simulink model "AlKaseeh_PhysicalTwin_PM_FinalScientific_v4_6_2"  (R2025b)
settings: Solver=ode15s  StartTime=0.0  StopTime=9000  MaxStep=0.1  RelTol=1e-4
libraries: fl_lib x34, nesl_utility x24, ee_lib x1, slpidlib x1, SimscapeFluids_lib x1
(part 1 of 2)
settings Model: Creator=Iman.Hindi  LastModifiedBy=Iman.Hindi

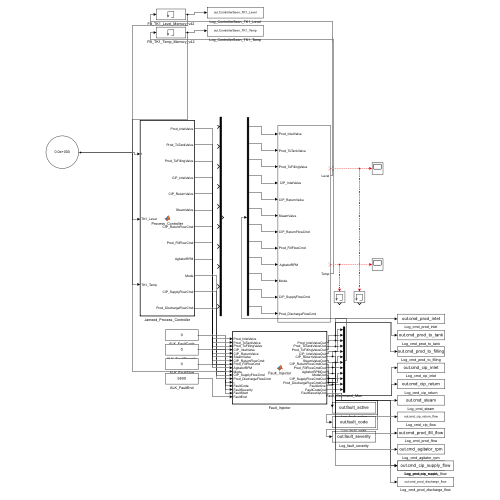
[thumbnail: Simulink's stored preview of the top-level diagram]
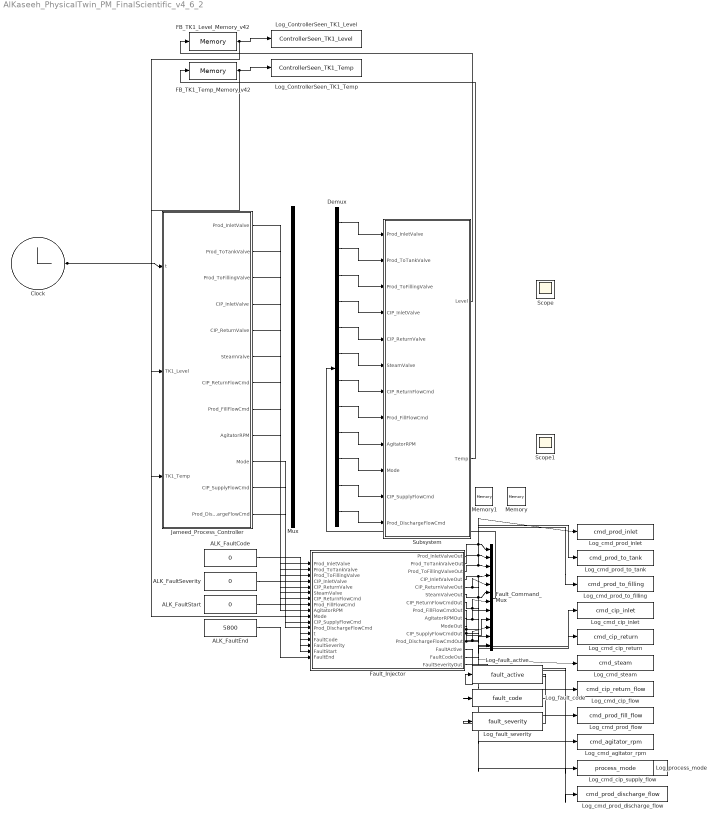
== system AlKaseeh_PhysicalTwin_PM_FinalScientific_v4_6_2 ==
  ALK_FaultCode : Constant  Value=0
  ALK_FaultEnd : Constant  Value=5800
  ALK_FaultSeverity : Constant  Value=0
  ALK_FaultStart : Constant  Value=0
  Clock : Clock
  Demux : Demux  Outputs=12
  FB_TK1_Level_Memory_v42 : Memory  InitialCondition=0.2
  FB_TK1_Temp_Memory_v42 : Memory  InitialCondition=300
  Fault_Command_Mux : Mux  Inputs=12
  Fault_Injector : MATLAB Function  TreatAsAtomicUnit=on
  Jameed_Process_Controller : MATLAB Function  TreatAsAtomicUnit=on
  Log_ControllerSeen_TK1_Level : ToWorkspace  VariableName=ControllerSeen_TK1_Level  SaveFormat=Timeseries  SampleTime=-1
  Log_ControllerSeen_TK1_Temp : ToWorkspace  VariableName=ControllerSeen_TK1_Temp  SaveFormat=Timeseries  SampleTime=-1
  Log_cmd_agitator_rpm : ToWorkspace  VariableName=cmd_agitator_rpm  SaveFormat=Timeseries  SampleTime=-1
  Log_cmd_cip_flow : ToWorkspace  VariableName=cmd_cip_return_flow  SaveFormat=Timeseries  SampleTime=-1
  Log_cmd_cip_inlet : ToWorkspace  VariableName=cmd_cip_inlet  SaveFormat=Timeseries  SampleTime=-1
  Log_cmd_cip_return : ToWorkspace  VariableName=cmd_cip_return  SaveFormat=Timeseries  SampleTime=-1
  Log_cmd_cip_supply_flow : ToWorkspace  VariableName=cmd_cip_supply_flow  SaveFormat=Timeseries  SampleTime=-1
  Log_cmd_prod_discharge_flow : ToWorkspace  VariableName=cmd_prod_discharge_flow  SaveFormat=Timeseries  SampleTime=-1
  Log_cmd_prod_flow : ToWorkspace  VariableName=cmd_prod_fill_flow  SaveFormat=Timeseries  SampleTime=-1
  Log_cmd_prod_inlet : ToWorkspace  VariableName=cmd_prod_inlet  SaveFormat=Timeseries  SampleTime=-1
  Log_cmd_prod_to_filling : ToWorkspace  VariableName=cmd_prod_to_filling  SaveFormat=Timeseries  SampleTime=-1
  Log_cmd_prod_to_tank : ToWorkspace  VariableName=cmd_prod_to_tank  SaveFormat=Timeseries  SampleTime=-1
  Log_cmd_steam : ToWorkspace  VariableName=cmd_steam  SaveFormat=Timeseries  SampleTime=-1
  Log_fault_active : ToWorkspace  VariableName=fault_active  SaveFormat=Timeseries  SampleTime=-1
  Log_fault_code : ToWorkspace  VariableName=fault_code  SaveFormat=Timeseries  SampleTime=-1
  Log_fault_severity : ToWorkspace  VariableName=fault_severity  SaveFormat=Timeseries  SampleTime=-1
  Log_process_mode : ToWorkspace  VariableName=process_mode  SaveFormat=Timeseries  SampleTime=-1
  Memory : Memory  InitialCondition=1
  Memory1 : Memory  InitialCondition=1
  Mux : Mux  Inputs=10
  Scope : Scope
  Scope1 : Scope
  Subsystem : Subsystem
  wires:
  ? -> Scope/1, Memory/1
  ? -> Scope1/1, Memory1/1
  Clock/1 -> Jameed_Process_Controller/1(t), Fault_Injector/13(t)
  Jameed_Process_Controller/1(Prod_InletValve) -> Fault_Injector/1(Prod_InletValve)
  Jameed_Process_Controller/2(Prod_ToTankValve) -> Fault_Injector/2(Prod_ToTankValve)
  Jameed_Process_Controller/3(Prod_ToFillingValve) -> Fault_Injector/3(Prod_ToFillingValve)
  Jameed_Process_Controller/4(CIP_InletValve) -> Fault_Injector/4(CIP_InletValve)
  Jameed_Process_Controller/5(CIP_ReturnValve) -> Fault_Injector/5(CIP_ReturnValve)
  Jameed_Process_Controller/6(SteamValve) -> Fault_Injector/6(SteamValve)
  Jameed_Process_Controller/7(CIP_ReturnFlowCmd) -> Fault_Injector/7(CIP_ReturnFlowCmd)
  Jameed_Process_Controller/8(Prod_FillFlowCmd) -> Fault_Injector/8(Prod_FillFlowCmd)
  Jameed_Process_Controller/9(AgitatorRPM) -> Fault_Injector/9(AgitatorRPM)
  Jameed_Process_Controller/10(Mode) -> Fault_Injector/10(Mode)
  Fault_Injector/1(Prod_InletValveOut) -> Fault_Command_Mux/1, Log_cmd_prod_inlet/1
  Fault_Injector/2(Prod_ToTankValveOut) -> Fault_Command_Mux/2, Log_cmd_prod_to_tank/1
  Fault_Injector/3(Prod_ToFillingValveOut) -> Fault_Command_Mux/3, Log_cmd_prod_to_filling/1
  Fault_Injector/4(CIP_InletValveOut) -> Fault_Command_Mux/4, Log_cmd_cip_inlet/1
  Fault_Injector/5(CIP_ReturnValveOut) -> Fault_Command_Mux/5, Log_cmd_cip_return/1
  Fault_Injector/6(SteamValveOut) -> Fault_Command_Mux/6, Log_cmd_steam/1
  Fault_Injector/7(CIP_ReturnFlowCmdOut) -> Fault_Command_Mux/7, Log_cmd_cip_flow/1
  Fault_Injector/8(Prod_FillFlowCmdOut) -> Fault_Command_Mux/8, Log_cmd_prod_flow/1
  Fault_Injector/9(AgitatorRPMOut) -> Fault_Command_Mux/9, Log_cmd_agitator_rpm/1
  Fault_Injector/10(ModeOut) -> Fault_Command_Mux/10, Log_process_mode/1
  Fault_Command_Mux/1 -> Demux/1
  Jameed_Process_Controller/11(CIP_SupplyFlowCmd) -> Fault_Injector/11(CIP_SupplyFlowCmd)
  Jameed_Process_Controller/12(Prod_DischargeFlowCmd) -> Fault_Injector/12(Prod_DischargeFlowCmd)
  ALK_FaultCode/1 -> Fault_Injector/14(FaultCode)
  ALK_FaultSeverity/1 -> Fault_Injector/15(FaultSeverity)
  ALK_FaultStart/1 -> Fault_Injector/16(FaultStart)
  ALK_FaultEnd/1 -> Fault_Injector/17(FaultEnd)
  Fault_Injector/11(CIP_SupplyFlowCmdOut) -> Fault_Command_Mux/11, Log_cmd_cip_supply_flow/1
  Fault_Injector/12(Prod_DischargeFlowCmdOut) -> Fault_Command_Mux/12, Log_cmd_prod_discharge_flow/1
  Fault_Injector/13(FaultActive) -> Log_fault_active/1
  Fault_Injector/14(FaultCodeOut) -> Log_fault_code/1
  Fault_Injector/15(FaultSeverityOut) -> Log_fault_severity/1
  Demux/1 -> Subsystem/1(Prod_InletValve)
  Demux/2 -> Subsystem/2(Prod_ToTankValve)
  Demux/3 -> Subsystem/3("Prod_ToFillingValve ")
  Demux/4 -> Subsystem/4(" CIP_InletValve")
  Demux/5 -> Subsystem/5(CIP_ReturnValve)
  Demux/6 -> Subsystem/6(SteamValve)
  Demux/7 -> Subsystem/7(CIP_ReturnFlowCmd)
  Demux/8 -> Subsystem/8(Prod_FillFlowCmd)
  Demux/9 -> Subsystem/9(" AgitatorRPM")
  Demux/10 -> Subsystem/10(Mode)
  Demux/11 -> Subsystem/11(CIP_SupplyFlowCmd)
  Demux/12 -> Subsystem/12(Prod_DischargeFlowCmd)
  Subsystem/1(Level) -> FB_TK1_Level_Memory_v42/1
  Subsystem/2(Temp) -> FB_TK1_Temp_Memory_v42/1
  FB_TK1_Level_Memory_v42/1 -> Jameed_Process_Controller/2(TK1_Level), Log_ControllerSeen_TK1_Level/1
  FB_TK1_Temp_Memory_v42/1 -> Jameed_Process_Controller/3(TK1_Temp), Log_ControllerSeen_TK1_Temp/1

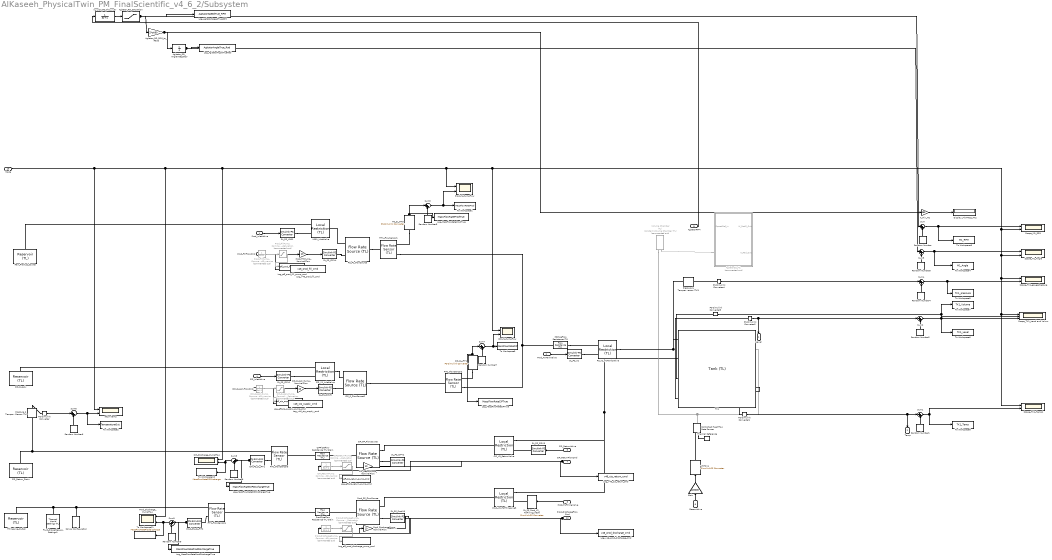
== system AlKaseeh_PhysicalTwin_PM_FinalScientific_v4_6_2/Subsystem ==
  Prod_InletValve : Inport
  Prod_ToTankValve : Inport  Port=2
  "Prod_ToFillingValve " : Inport  Port=3
  " CIP_InletValve" : Inport  Port=4
  CIP_ReturnValve : Inport  Port=5
  SteamValve : Inport  Port=6
  CIP_ReturnFlowCmd : Inport  Port=7
  Prod_FillFlowCmd : Inport  Port=8
  " AgitatorRPM" : Inport  Port=9
  Mode : Inport  Port=10
  CIP_SupplyFlowCmd : Inport  Port=11
  Prod_DischargeFlowCmd : Inport  Port=12
  AgitatorSS_M1 : Subsystem  Commented=on
      mask help:
      | Agitator Electromechanical Model
      | Speed ref (RPM) → rad/s → Ideal Velocity Source
      | Measures angular velocity W (rad/s) and angle A (rad)
      | Nominal speed: 23.3 RPM = 2.440 rad/s
      | IL coupling: W output → mixing pressure = 965 × W Pa
  Agitator_RO_AngleIntegrator : Integrator
  Agitator_RO_FirstOrder : TransferFcn  Numerator=1  Denominator=[3 1]
  Agitator_RO_RPM_to_RadS : Gain  Gain=2*pi/60
  Agitator_RO_Saturation : Saturate  UpperLimit=30  LowerLimit=0
  CIPPipeFlow Resistance (TL) drain : fl_lib/Thermal Liquid/Elements/Flow Resistance (TL)  delta_p_nominal=0.001 MPa  mdot_nominal=10 kg/s  area=0.01 m^2  laminar_fraction=1e-3
  CIP_Discharge_PumpFlow : Scope  NumInputPorts=2
      settings: ActiveDisplayYMinimum=-1.4917140570231822  ActiveDisplayYMaximum=11.439960668136928  DataLoggingVariableName=ScopeData3
  CIP_IN_PumpFlow : Scope  NumInputPorts=2
      settings: ActiveDisplayYMinimum=-1.4917140570231822  ActiveDisplayYMaximum=11.439960668136928  DataLoggingVariableName=ScopeData2
  CIP_PS_SL_FIT1 : nesl_utility/PS-Simulink Converter  PhysicalDomain=network_engine_domain  SubClassName=ps_output  LeftPortType=input  RightPortType=output  PseudoPeriodic=off  Frequencies=[]  VectorFormat=inherit  Unit=inherit  AffineConversion=off
  CIP_P_FlowSource2 : fl_lib/Thermal Liquid/Sources/Flow Rate Source (TL)  source_type=foundation.enum.constant_controlled.controlled  flow_type=foundation.enum.mass_volumetric_flow.mass  mass_flow=0 kg/s  volumetric_flow=0 m^3/s  power_spec=foundation.enum.power_spec.none  area=0.01 m^2
  CIP_RP_FlowSource : fl_lib/Thermal Liquid/Sources/Flow Rate Source (TL)  source_type=foundation.enum.constant_controlled.controlled  flow_type=foundation.enum.mass_volumetric_flow.mass  mass_flow=0 kg/s  volumetric_flow=0 m^3/s  power_spec=foundation.enum.power_spec.none  area=0.01 m^2
  CIP_ReturnPump_CommandDynamics : TransferFcn  Commented=on  Numerator=1  Denominator=[5 1]
  CIP_ReturnPump_CommandDynamics_Saturation : Saturate  Commented=on  UpperLimit=1  LowerLimit=0
  CIP_ReturnPump_NominalFlow : Gain  Gain=10
  CIP_Return_Drain : fl_lib/Thermal Liquid/Elements/Reservoir (TL)  pressure_spec=foundation.enum.pressure_spec.atmospheric  reservoir_pressure=0.101325 MPa  reservoir_temperature=300 K  area=0.01 m^2
  CIP_SL_FIT1 : nesl_utility/PS-Simulink Converter  PhysicalDomain=network_engine_domain  SubClassName=ps_output  LeftPortType=input  RightPortType=output  PseudoPeriodic=off  Frequencies=[]  VectorFormat=inherit  Unit=inherit  AffineConversion=off
  CIP_Supply : fl_lib/Thermal Liquid/Elements/Reservoir (TL)  pressure_spec=foundation.enum.pressure_spec.atmospheric  reservoir_pressure=0.101325 MPa  reservoir_temperature=300 K  area=0.01 m^2
  CIP_SupplyPump_CommandDynamics : TransferFcn  Commented=on  Numerator=1  Denominator=[5 1]
  CIP_SupplyPump_CommandDynamics_Saturation : Saturate  Commented=on  UpperLimit=1  LowerLimit=0
  CIP_SupplyPump_NominalFlow : Gain  Gain=10
  CIP_V1_InletValve : fl_lib/Thermal Liquid/Elements/Local Restriction (TL)  restriction_type=foundation.enum.restriction_type.variable  restriction_area=0.001 m^2  min_area=1e-10 m^2  max_area=0.005 m^2  area=0.01 m^2  Cd=0.64  Re_c=150  pressure_recovery=true
      settings: InternalSimscapePortConfiguration="{\"Bottom\":[],\"Left\":[{\"id\":\"A\",\"label\":\"A\",\"type\":\"foundation.thermal_liquid.thermal_liquid\"},{\"id\":\"area_in\",\"label\":\"AR\",\"type\":\"input\"}],\"Right\":[{\"id\":\"B\",\"label\":\"B\",\"type\":\"foundation.thermal_liquid.thermal_liquid\"}],\"Top\":[]}"
  CIP_V3_ReturnValve : fl_lib/Thermal Liquid/Elements/Local Restriction (TL)  restriction_type=foundation.enum.restriction_type.variable  restriction_area=0.001 m^2  min_area=1e-10 m^2  max_area=0.005 m^2  area=0.01 m^2  Cd=0.64  Re_c=150  pressure_recovery=true
      settings: InternalSimscapePortConfiguration="{\"Bottom\":[],\"Left\":[{\"id\":\"A\",\"label\":\"A\",\"type\":\"foundation.thermal_liquid.thermal_liquid\"},{\"id\":\"area_in\",\"label\":\"AR\",\"type\":\"input\"}],\"Right\":[{\"id\":\"B\",\"label\":\"B\",\"type\":\"foundation.thermal_liquid.thermal_liquid\"}],\"Top\":[]}"
  Controlled Heat Flow Rate Source : fl_lib/Thermal/Thermal Sources/Controlled Heat Flow Rate Source
  Display_MixPress_TK2 : Display
  FIT1_FlowSensor{1..4} (4 alike) : fl_lib/Thermal Liquid/Sensors/Flow Rate Sensor (TL)  mass_flow_measure=true  volumetric_flow_measure=false  energy_flow_measure=false
      settings: InternalSimscapePortConfiguration="{\"Bottom\":[],\"Left\":[{\"id\":\"A\",\"label\":\"A\",\"type\":\"foundation.thermal_liquid.thermal_liquid\"}],\"Right\":[{\"id\":\"B\",\"label\":\"B\",\"type\":\"foundation.thermal_liquid.thermal_liquid\"},{\"id\":\"M\",\"label\":\"M\",\"type\":\"output\"}],\"Top\":[]}"
  FillingLine_Outlet : fl_lib/Thermal Liquid/Elements/Reservoir (TL)  pressure_spec=foundation.enum.pressure_spec.atmospheric  reservoir_pressure=0.101325 MPa  reservoir_temperature=300 K  area=0.01 m^2
  Fluid_Properties_or_Settings1 : fl_lib/Thermal Liquid/Utilities/Thermal Liquid Settings (TL)  table_dimensions=foundation.enum.table_dimensions_TL.one_dimensional  T_TLU=[273.16, 335, 340, 343] K  p_TLU=[0.01, 0.1, 5 : 5 : 50] MPa  p_atm=0.101325 MPa  pT_region_flag=foundation.enum.pT_region_TL.min_max  T_min=273.16 K  T_max=373.16 K  p_min=0.01 MPa  p_max=50 MPa  T_min_1D=273.16 K  T_max_1D=343 K  p_min_1D=0.01 MPa  p_max_1D=50 MPa  pT_validity_TLU=[1, 1, 1, 1, 1, 1, 1, 1, 1, 1, 1, 1; 1, 1, 1, 1, 1, 1, 1, 1, 1, 1, 1, 1; 1, 1, 1, 1, 1, 1, 1, 1, 1, 1, 1, 1; 1, 1, 1, 1, 1, 1, 1, 1, 1, 1, 1, 1; 1, 1, 1, 1, 1, 1, 1, 1, 1, 1, 1, 1; 0, 1, 1, 1, 1, 1, 1, 1, 1, 1, 1, 1; 0, 1, 1, 1, 1, 1, 1, 1, 1, 1, 1, 1; 0, 1, 1, 1, 1, 1, 1, 1, 1, 1, 1, 1; 0, 1, 1, 1, 1, 1, 1, 1, 1, 1, 1, 1; 0, 1, 1, 1, 1, 1, 1, 1, 1, 1, 1, 1; 0, 0, 1, 1, 1, 1, 1, 1, 1, 1, 1, 1]  properties_range_check=simscape.enum.assert.action.warn  rho_parameterization_2D=foundation.enum.rho_parameterization_2D.rho_beta_alpha  rho_parameterization_1D=foundation.enum.rho_parameterization_1D.rho_vector  rho_TLU=1100 kg/m^3  beta_TLU=[1.9649, 1.9654, 1.9929, 2.0213, 2.0499, 2.0787, 2.1078, 2.1372, 2.1668, 2.1966, 2.2268, 2.2572; 2.0913, 2.0918, 2.1191, 2.1471, 2.1752, 2.2036, 2.2322, 2.261, 2.2899, 2.3191, 2.3485, 2.3781; 2.1786, 2.1791, 2.2067, 2.235, 2.2634, 2.2919, 2.3206, 2.3494, 2.3784, 2.4075, 2.4367, 2.4661; 2.2332, 2.2337, 2.2619, 2.2908, 2.3197, 2.3487, 2.3778, 2.407, 2.4363, 2.4657, 2.4951, 2.5246; 2.26, 2.2605, 2.2895, 2.3191, 2.3487, 2.3784, 2.4081, 2.4378, 2.4675, 2.4973, 2.5272, 2.5571; 2.2638, 2.2638, 2.2936, 2.324, 2.3544, 2.3848, 2.4151, 2.4455, 2.4758, 2.5062, 2.5365, 2.5669; 2.2472, 2.2472, 2.2779, 2.3092, 2.3403, 2.3715, 2.4025, 2.4336, 2.4646, 2.4955, 2.5264, 2.5573; 2.214, 2.214, 2.2455, 2.2776, 2.3096, 2.3415, 2.3733, 2.405, 2.4367, 2.4683, 2.4998, 2.5313; 2.1668, 2.1668, 2.1992, 2.2321, 2.2649, 2.2976, 2.3301, 2.3626, 2.3949, 2.4272, 2.4593, 2.4914; 2.1081, 2.1081, 2.1413, 2.175, 2.2086, 2.2421, 2.2754, 2.3085, 2.3415, 2.3744, 2.4072, 2.4399; 2.0494, 2.0494, 2.0739, 2.1084, 2.1428, 2.177, 2.211, 2.2449, 2.2786, 2.3121, 2.3455, 2.3788] GPa  alpha_TLU=1e-4 * [-.679, -.676, -.49, -.307, -.13, .041, .206, .365, .519, .668, .811, .949; .878, .881, .998, 1.114, 1.227, 1.337, 1.445, 1.549, 1.651, 1.75, 1.846, 1.939; 2.068, 2.069, 2.141, 2.213, 2.283, 2.352, 2.42, 2.486, 2.551, 2.614, 2.676, 2.736; 3.034, 3.035, 3.074, 3.113, 3.152, 3.191, 3.229, 3.267, 3.305, 3.341, 3.377, 3.413; 3.855, 3.856, 3.87, 3.884, 3.899, 3.914, 3.93, 3.946, 3.961, 3.977, 3.993, 4.009; 4.578, 4.578, 4.572, 4.566, 4.562, 4.558, 4.555, 4.552, 4.55, 4.549, 4.548, 4.547; 5.233, 5.233, 5.209, 5.186, 5.165, 5.144, 5.125, 5.107, 5.09, 5.074, 5.059, 5.045; 5.84, 5.84, 5.801, 5.762, 5.725, 5.691, 5.657, 5.625, 5.595, 5.566, 5.538, 5.512; 6.414, 6.414, 6.36, 6.307, 6.256, 6.208, 6.161, 6.117, 6.074, 6.033, 5.994, 5.956; 6.967, 6.967, 6.898, 6.831, 6.766, 6.705, 6.646, 6.589, 6.535, 6.482, 6.432, 6.384; 7.519, 7.519, 7.423, 7.342, 7.264, 7.189, 7.118, 7.049, 6.983, 6.92, 6.859, 6.8] 1/K  rho_TLU_2=[999.7973, 999.8431, 1002.3216, 1004.8218, 1007.293, 1009.7358, 1012.1506, 1014.5379, 1016.8979, 1019.2311, 1021.538, 1023.8188; 999.6579, 999.7009, 1002.0303, 1004.382, 1006.7084, 1009.0101, 1011.2874, 1013.5407, 1015.7703, 1017.9766, 1020.1599, 1022.3206; 998.1632, 998.2045, 1000.4375, 1002.6924, 1004.9239, 1007.1324, 1009.3183, 1011.4819, 1013.6236, 1015.7438, 1017.8428, 1019.921; 995.6057, 995.6458, 997.81864, 1000.0128, 1002.1841, 1004.3332, 1006.4603, 1008.566, 1010.6505, 1012.7144, 1014.758, 1016.7815; 992.1724, 992.2119, 994.3513, 996.5113, 998.6484, 1000.7633, 1002.8563, 1004.928, 1006.9788, 1009.009, 1011.0192, 1013.0097; 988.02, 988.0299, 990.1568, 992.3035, 994.4268, 996.5273, 998.6056, 1000.6622, 1002.6976, 1004.7123, 1006.7067, 1008.6813; 983.18, 983.1901, 985.3217, 987.4721, 989.5983, 991.7008, 993.7803, 995.8374, 997.8726, 999.8864, 1001.8795, 1003.8522; 977.75, 977.7583, 979.9094, 982.0783, 984.2216, 986.34, 988.4343, 990.505, 992.5529, 994.5786, 996.5825, 998.5654; 971.77, 971.7836, 973.9673, 976.1678, 978.3409, 980.4876, 982.6087, 984.7049, 986.7768, 988.8254, 990.8511, 992.8545; 965.26, 965.3023, 967.5311, 969.7753, 971.9901, 974.1764, 976.3354, 978.4676, 980.5741, 982.6556, 984.7129, 986.7465; 958.62, 958.6315, 960.627, 962.9267, 965.1944, 967.4314, 969.6387, 971.8173, 973.9681, 976.0921, 978.19, 980.2628] kg/m^3  rho_ref_3=998.21 kg/m^3  T_ref_3=293.16 K  p_ref_3=0.101325 MPa  beta_const_3=2.1791 GPa  alpha_const_3=2.0691e-4 1/K  rho_TLU_4=[1100, 1100, 1100, 1100] kg/m^3  beta_const_4=2.1791 GPa  p_ref_4=0.101325 MPa  rho_ref_5=998.21 kg/m^3  T_ref_5=293.16 K  p_ref_5=0.101325 MPa  beta_const_5=2.1791 GPa  alpha_const_5=2.0691e-4 1/K  u_parameterization_2D=foundation.enum.u_parameterization_2D.u_cp  u_parameterization_1D=foundation.enum.u_parameterization_1D.u  u_TLU=[.0002, .0018, .086, .1588, .219, .267, .3034, .3288, .3436, .3483, .3435, .3294; 42.062, 42.06, 41.935, 41.804, 41.668, 41.527, 41.382, 41.233, 41.081, 40.924, 40.763, 40.599; 83.953, 83.948, 83.651, 83.349, 83.049, 82.749, 82.451, 82.153, 81.856, 81.56, 81.265, 80.971; 125.77, 125.76, 125.31, 124.86, 124.41, 123.97, 123.53, 123.1, 122.68, 122.25, 121.84, 121.42; 167.57, 167.56, 166.96, 166.37, 165.79, 165.21, 164.65, 164.09, 163.54, 163, 162.46, 161.94; 209.36, 209.36, 208.63, 207.9, 207.19, 206.48, 205.79, 205.11, 204.45, 203.79, 203.14, 202.5; 251.19, 251.19, 250.33, 249.47, 248.62, 247.79, 246.98, 246.18, 245.39, 244.62, 243.86, 243.12; 293.06, 293.06, 292.07, 291.07, 290.1, 289.14, 288.2, 287.28, 286.38, 285.49, 284.62, 283.77; 334.99, 334.99, 333.86, 332.73, 331.63, 330.54, 329.48, 328.44, 327.41, 326.41, 325.43, 324.46; 377, 377, 375.73, 374.46, 373.22, 372, 370.81, 369.64, 368.5, 367.38, 366.27, 365.19; 419.01, 419.01, 417.69, 416.27, 414.89, 413.54, 412.21, 410.91, 409.64, 408.4, 407.17, 405.98] kJ/kg  cp_TLU=[4.2199, 4.2194, 4.1957, 4.1726, 4.1508, 4.13, 4.1103, 4.0916, 4.0738, 4.0569, 4.0408, 4.0254; 4.1955, 4.1951, 4.1769, 4.1592, 4.1422, 4.1259, 4.1103, 4.0954, 4.0812, 4.0676, 4.0545, 4.0421; 4.1843, 4.184, 4.169, 4.1543, 4.1401, 4.1264, 4.1133, 4.1007, 4.0885, 4.0768, 4.0656, 4.0548; 4.1801, 4.1798, 4.1667, 4.1538, 4.1413, 4.1293, 4.1177, 4.1064, 4.0956, 4.0851, 4.075, 4.0653; 4.1796, 4.1794, 4.1675, 4.1558, 4.1444, 4.1334, 4.1227, 4.1123, 4.1023, 4.0926, 4.0832, 4.0741; 4.1813, 4.1813, 4.1702, 4.1592, 4.1484, 4.138, 4.1279, 4.1181, 4.1086, 4.0993, 4.0903, 4.0816; 4.185, 4.185, 4.1742, 4.1636, 4.1532, 4.1432, 4.1334, 4.1239, 4.1146, 4.1056, 4.0969, 4.0884; 4.1901, 4.1901, 4.1795, 4.169, 4.1588, 4.1489, 4.1393, 4.1299, 4.1207, 4.1118, 4.1032, 4.0947; 4.1968, 4.1968, 4.1862, 4.1757, 4.1655, 4.1555, 4.1458, 4.1364, 4.1273, 4.1183, 4.1096, 4.1012; 4.2052, 4.2052, 4.1944, 4.1837, 4.1733, 4.1632, 4.1534, 4.1438, 4.1345, 4.1255, 4.1166, 4.108; 4.2136, 4.2136, 4.2045, 4.1935, 4.1828, 4.1724, 4.1623, 4.1524, 4.1429, 4.1335, 4.1245, 4.1157] kJ/(K*kg)  u_TLU_2=[.0002, .0018, .086, .1588, .219, .267, .3034, .3288, .3436, .3483, .3435, .3294; 42.062, 42.06, 41.935, 41.804, 41.668, 41.527, 41.382, 41.233, 41.081, 40.924, 40.763, 40.599; 83.953, 83.948, 83.651, 83.349, 83.049, 82.749, 82.451, 82.153, 81.856, 81.56, 81.265, 80.971; 125.77, 125.76, 125.31, 124.86, 124.41, 123.97, 123.53, 123.1, 122.68, 122.25, 121.84, 121.42; 167.57, 167.56, 166.96, 166.37, 165.79, 165.21, 164.65, 164.09, 163.54, 163, 162.46, 161.94; 209.36, 209.36, 208.63, 207.9, 207.19, 206.48, 205.79, 205.11, 204.45, 203.79, 203.14, 202.5; 251.19, 251.19, 250.33, 249.47, 248.62, 247.79, 246.98, 246.18, 245.39, 244.62, 243.86, 243.12; 293.06, 293.06, 292.07, 291.07, 290.1, 289.14, 288.2, 287.28, 286.38, 285.49, 284.62, 283.77; 334.99, 334.99, 333.86, 332.73, 331.63, 330.54, 329.48, 328.44, 327.41, 326.41, 325.43, 324.46; 377, 377, 375.73, 374.46, 373.22, 372, 370.81, 369.64, 368.5, 367.38, 366.27, 365.19; 419.01, 419.01, 417.69, 416.27, 414.89, 413.54, 412.21, 410.91, 409.64, 408.4, 407.17, 405.98] kJ/kg  cp_TLU_3=[4.2199, 4.2194, 4.1957, 4.1726, 4.1508, 4.13, 4.1103, 4.0916, 4.0738, 4.0569, 4.0408, 4.0254; 4.1955, 4.1951, 4.1769, 4.1592, 4.1422, 4.1259, 4.1103, 4.0954, 4.0812, 4.0676, 4.0545, 4.0421; 4.1843, 4.184, 4.169, 4.1543, 4.1401, 4.1264, 4.1133, 4.1007, 4.0885, 4.0768, 4.0656, 4.0548; 4.1801, 4.1798, 4.1667, 4.1538, 4.1413, 4.1293, 4.1177, 4.1064, 4.0956, 4.0851, 4.075, 4.0653; 4.1796, 4.1794, 4.1675, 4.1558, 4.1444, 4.1334, 4.1227, 4.1123, 4.1023, 4.0926, 4.0832, 4.0741; 4.1813, 4.1813, 4.1702, 4.1592, 4.1484, 4.138, 4.1279, 4.1181, 4.1086, 4.0993, 4.0903, 4.0816; 4.185, 4.185, 4.1742, 4.1636, 4.1532, 4.1432, 4.1334, 4.1239, 4.1146, 4.1056, 4.0969, 4.0884; 4.1901, 4.1901, 4.1795, 4.169, 4.1588, 4.1489, 4.1393, 4.1299, 4.1207, 4.1118, 4.1032, 4.0947; 4.1968, 4.1968, 4.1862, 4.1757, 4.1655, 4.1555, 4.1458, 4.1364, 4.1273, 4.1183, 4.1096, 4.1012; 4.2052, 4.2052, 4.1944, 4.1837, 4.1733, 4.1632, 4.1534, 4.1438, 4.1345, 4.1255, 4.1166, 4.108; 4.2136, 4.2136, 4.2045, 4.1935, 4.1828, 4.1724, 4.1623, 4.1524, 4.1429, 4.1335, 4.1245, 4.1157] kJ/(K*kg)  u_TLU_4=[0, 50, 100, 150] kJ/kg  cp_TLU_5=[4.2199; 4.1955; 4.1843; 4.1801; 4.1796; 4.1813; 4.185; 4.1901; 4.1968; 4.2052; 4.2136] kJ/(K*kg)  nu_TLU=8000 mm^2/s  nu_TLU_2=[8000, 8000, 8000, 8000] mm^2/s  k_TLU=[561.04, 561.09, 563.8, 566.56, 569.32, 572.08, 574.82, 577.54, 580.24, 582.92, 585.57, 588.18; 580.02, 580.07, 582.45, 584.88, 587.32, 589.75, 592.18, 594.61, 597.02, 599.42, 601.8, 604.16; 598.44, 598.48, 600.73, 603.03, 605.33, 607.64, 609.94, 612.24, 614.54, 616.82, 619.1, 621.36; 615.48, 615.52, 617.73, 620, 622.26, 624.54, 626.81, 629.07, 631.34, 633.6, 635.85, 638.09; 630.6, 630.64, 632.87, 635.15, 637.44, 639.72, 642.01, 644.29, 646.57, 648.84, 651.11, 653.36; 643.61, 643.61, 645.88, 648.21, 650.53, 652.86, 655.18, 657.51, 659.82, 662.14, 664.44, 666.74; 654.39, 654.39, 656.73, 659.12, 661.5, 663.89, 666.27, 668.65, 671.02, 673.38, 675.74, 678.09; 663.13, 663.13, 665.54, 668, 670.46, 672.91, 675.36, 677.8, 680.24, 682.67, 685.09, 687.5; 670.02, 670.02, 672.51, 675.05, 677.59, 680.12, 682.64, 685.16, 687.67, 690.17, 692.66, 695.14; 675.27, 675.27, 677.85, 680.48, 683.11, 685.73, 688.34, 690.94, 693.53, 696.11, 698.68, 701.24; 680.52, 680.52, 681.77, 684.5, 687.22, 689.94, 692.64, 695.34, 698.02, 700.69, 703.35, 706] mW/(K*m)  k_TLU_2=[560, 560, 560, 560] mW/(K*m)
  Gain : Gain  Gain=120000
  K_Mix_M2 : Gain  Gain=965
  Log_AgitatorAngleTrueRad : ToWorkspace  VariableName=AgitatorAngleTrue_Rad  SaveFormat=Timeseries  SampleTime=-1
  Log_AgitatorSpeedTrueRPM : ToWorkspace  VariableName=AgitatorSpeedTrue_RPM  SaveFormat=Timeseries  SampleTime=-1
  Log_MassFlowRateCIPDischargeTrue : ToWorkspace  VariableName=MassFlowRateCIPDischargeTrue  SaveFormat=Timeseries  SampleTime=-1
  Log_MassFlowRateCIPTrue : ToWorkspace  VariableName=MassFlowRateCIPTrue  SaveFormat=Timeseries  SampleTime=-1
  Log_MassFlowRateProdDischargeTrue : ToWorkspace  VariableName=MassFlowRateProdDischargeTrue  SaveFormat=Timeseries  SampleTime=-1
  Log_MassFlowRateProdTrue : ToWorkspace  VariableName=MassFlowRateProdTrue  SaveFormat=Timeseries  SampleTime=-1
  Log_eff_cip_return_pump_cmd : ToWorkspace  VariableName=eff_cip_return_pump_cmd  SaveFormat=Timeseries  SampleTime=-1
  Log_eff_cip_supply_pump_cmd : ToWorkspace  VariableName=eff_cip_supply_pump_cmd  SaveFormat=Timeseries  SampleTime=-1
  Log_eff_prod_discharge_pump_cmd : ToWorkspace  VariableName=eff_prod_discharge_pump_cmd  SaveFormat=Timeseries  SampleTime=-1
  Log_eff_prod_fill_pump_cmd : ToWorkspace  VariableName=eff_prod_fill_pump_cmd  SaveFormat=Timeseries  SampleTime=-1
  Log_v46_cip_return_cmd : ToWorkspace  VariableName=v46_cip_return_cmd  SaveFormat=Timeseries  SampleTime=-1
  Log_v46_cip_supply_cmd : ToWorkspace  VariableName=v46_cip_supply_cmd  SaveFormat=Timeseries  SampleTime=-1
  Log_v46_prod_discharge_cmd : ToWorkspace  VariableName=v46_prod_discharge_cmd  SaveFormat=Timeseries  SampleTime=-1
  Log_v46_prod_fill_cmd : ToWorkspace  VariableName=v46_prod_fill_cmd  SaveFormat=Timeseries  SampleTime=-1
  PS-Simulink Converter : nesl_utility/PS-Simulink Converter  PhysicalDomain=network_engine_domain  SubClassName=ps_output  LeftPortType=input  RightPortType=output  PseudoPeriodic=off  Frequencies=[]  VectorFormat=inherit  Unit=degC  AffineConversion=off
  PS-Simulink Converter{1..4} (4 alike) : nesl_utility/PS-Simulink Converter  PhysicalDomain=network_engine_domain  SubClassName=ps_output  LeftPortType=input  RightPortType=output  PseudoPeriodic=off  Frequencies=[]  VectorFormat=inherit  Unit=inherit  AffineConversion=off
  PSPipeFlow Resistance (TL) : fl_lib/Thermal Liquid/Elements/Flow Resistance (TL)  delta_p_nominal=0.1 MPa  mdot_nominal=10 kg/s  area=0.01 m^2  laminar_fraction=0.01
  PS_P1_FlowSource : fl_lib/Thermal Liquid/Sources/Flow Rate Source (TL)  source_type=foundation.enum.constant_controlled.controlled  flow_type=foundation.enum.mass_volumetric_flow.mass  mass_flow=0 kg/s  volumetric_flow=0 m^3/s  power_spec=foundation.enum.power_spec.none  area=0.01 m^2
  PS_SL_FIT3 : nesl_utility/PS-Simulink Converter  PhysicalDomain=network_engine_domain  SubClassName=ps_output  LeftPortType=input  RightPortType=output  PseudoPeriodic=off  Frequencies=[]  VectorFormat=inherit  Unit=inherit  AffineConversion=off
  PS_V2_ToTanksValve : fl_lib/Thermal Liquid/Elements/Local Restriction (TL)  restriction_type=foundation.enum.restriction_type.variable  restriction_area=0.001 m^2  min_area=1e-10 m^2  max_area=0.005 m^2  area=0.01 m^2  Cd=0.64  Re_c=150  pressure_recovery=true
      settings: InternalSimscapePortConfiguration="{\"Bottom\":[],\"Left\":[{\"id\":\"A\",\"label\":\"A\",\"type\":\"foundation.thermal_liquid.thermal_liquid\"},{\"id\":\"area_in\",\"label\":\"AR\",\"type\":\"input\"}],\"Right\":[{\"id\":\"B\",\"label\":\"B\",\"type\":\"foundation.thermal_liquid.thermal_liquid\"}],\"Top\":[]}"
  Pressure & Temperature Sensor (TL) : fl_lib/Thermal Liquid/Sensors/Pressure & Temperature Sensor (TL)  reference=foundation.enum.MeasurementReference.absolute  pressure=false  pressure_spec=foundation.enum.PressureMeasementSpec.Absolute  temperature=true
      settings: InternalSimscapePortConfiguration="{\"Bottom\":[{\"id\":\"T\",\"label\":\"T\",\"type\":\"output\"}],\"Left\":[{\"id\":\"A\",\"label\":\"A\",\"type\":\"foundation.thermal_liquid.thermal_liquid\"}],\"Right\":[],\"Top\":[]}"
  Pressure & Temperature Sensor (TL)1 : fl_lib/Thermal Liquid/Sensors/Pressure & Temperature Sensor (TL)  reference=foundation.enum.MeasurementReference.absolute  pressure=true  pressure_spec=foundation.enum.PressureMeasementSpec.Gauge  temperature=false
      settings: InternalSimscapePortConfiguration="{\"Bottom\":[],\"Left\":[{\"id\":\"A\",\"label\":\"A\",\"type\":\"foundation.thermal_liquid.thermal_liquid\"}],\"Right\":[{\"id\":\"Pg\",\"label\":\"Pg\",\"type\":\"output\"}],\"Top\":[]}"
  ProdPipeFlow Resistance (TL) drain : fl_lib/Thermal Liquid/Elements/Flow Resistance (TL)  delta_p_nominal=0.001 MPa  mdot_nominal=10 kg/s  area=0.01 m^2  laminar_fraction=1e-3
  Prod_DischargePump_CommandDynamics : TransferFcn  Commented=on  Numerator=1  Denominator=[3 1]
  Prod_DischargePump_CommandDynamics_Saturation : Saturate  Commented=on  UpperLimit=1  LowerLimit=0
  Prod_DischargePump_NominalFlow : Gain  Gain=10
  Prod_Discharge_PumpFlow : Scope  NumInputPorts=2
      settings: ActiveDisplayYMinimum=-1.4917140570231822  ActiveDisplayYMaximum=11.439960668136928  DataLoggingVariableName=ScopeData9
  Prod_FillPump_CommandDynamics : TransferFcn  Commented=on  Numerator=1  Denominator=[2 1]
  Prod_FillPump_CommandDynamics_Saturation : Saturate  Commented=on  UpperLimit=1  LowerLimit=0
  Prod_FillPump_NominalFlow : Gain  Gain=10
  Prod_IN_PumpFlow : Scope  NumInputPorts=2
      settings: ActiveDisplayYMinimum=-1.4917140570231822  ActiveDisplayYMaximum=11.439960668136928  DataLoggingVariableName=ScopeData6
  Prod_PS_SL_FIT2 : nesl_utility/PS-Simulink Converter  PhysicalDomain=network_engine_domain  SubClassName=ps_output  LeftPortType=input  RightPortType=output  PseudoPeriodic=off  Frequencies=[]  VectorFormat=inherit  Unit=inherit  AffineConversion=off
  Prod_RP_FlowSource : fl_lib/Thermal Liquid/Sources/Flow Rate Source (TL)  source_type=foundation.enum.constant_controlled.controlled  flow_type=foundation.enum.mass_volumetric_flow.mass  mass_flow=0 kg/s  volumetric_flow=0 m^3/s  power_spec=foundation.enum.power_spec.none  area=0.01 m^2
  Prod_V2_ToFillingLine3 : fl_lib/Thermal Liquid/Elements/Local Restriction (TL)  restriction_type=foundation.enum.restriction_type.variable  restriction_area=0.001 m^2  min_area=1e-10 m^2  max_area=0.005 m^2  area=0.01 m^2  Cd=0.64  Re_c=150  pressure_recovery=true
      settings: InternalSimscapePortConfiguration="{\"Bottom\":[],\"Left\":[{\"id\":\"A\",\"label\":\"A\",\"type\":\"foundation.thermal_liquid.thermal_liquid\"},{\"id\":\"area_in\",\"label\":\"AR\",\"type\":\"input\"}],\"Right\":[{\"id\":\"B\",\"label\":\"B\",\"type\":\"foundation.thermal_liquid.thermal_liquid\"}],\"Top\":[]}"
  Random Number : RandomNumber  Variance=0.01  Seed=105  SampleTime=0.1
  Random Number1 : RandomNumber  Variance=0.0225  Seed=101  SampleTime=0.1
  Random Number2 : RandomNumber  Variance=4e-6  Seed=102  SampleTime=0.1
  Random Number{3,7..9} (4 alike) : RandomNumber  Variance=0.0025  Seed=103  SampleTime=0.1
  Random Number4 : RandomNumber  Variance=625  Seed=104  SampleTime=0.1
  Random Number5 : RandomNumber  Mean=0.00873  Variance=7.62e-5  Seed=107  SampleTime=0.1
  Random Number6 : RandomNumber  Variance=0.0225  Seed=106  SampleTime=0.1
  Raw_Product_Source : fl_lib/Thermal Liquid/Elements/Reservoir (TL)  pressure_spec=foundation.enum.pressure_spec.atmospheric  reservoir_pressure=0.101325 MPa  reservoir_temperature=300 K  area=0.01 m^2
  SL_PS_CIPV1 : nesl_utility/Simulink-PS Converter  PhysicalDomain=network_engine_domain  SubClassName=ps_input  LeftPortType=input  RightPortType=output  PseudoPeriodic=off  Frequencies=[]  NoiseDistribution=none  NoiseParameters=[]  Unit=1  AffineConversion=off  FilteringAndDerivatives=provide  SimscapeFilterOrder=1  InputFilterTimeConstant=0.001  UdotUserProvided=0
  SL_PS_CIPV2 : nesl_utility/Simulink-PS Converter  PhysicalDomain=network_engine_domain  SubClassName=ps_input  LeftPortType=input  RightPortType=output  PseudoPeriodic=off  Frequencies=[]  NoiseDistribution=none  NoiseParameters=[]  Unit=kg/s  AffineConversion=off  FilteringAndDerivatives=provide  SimscapeFilterOrder=1  InputFilterTimeConstant=0.001  UdotUserProvided=0
  SL_PS_CIPV3 : nesl_utility/Simulink-PS Converter  PhysicalDomain=network_engine_domain  SubClassName=ps_input  LeftPortType=input  RightPortType=output  PseudoPeriodic=off  Frequencies=[]  NoiseDistribution=none  NoiseParameters=[]  Unit=1  AffineConversion=off  FilteringAndDerivatives=provide  SimscapeFilterOrder=1  InputFilterTimeConstant=0.001  UdotUserProvided=0
  SL_PS_CIPV4 : nesl_utility/Simulink-PS Converter  PhysicalDomain=network_engine_domain  SubClassName=ps_input  LeftPortType=input  RightPortType=output  PseudoPeriodic=off  Frequencies=[]  NoiseDistribution=none  NoiseParameters=[]  Unit=kg/s  AffineConversion=off  FilteringAndDerivatives=provide  SimscapeFilterOrder=1  InputFilterTimeConstant=0.001  UdotUserProvided=0
  SL_PS_CIPV5 : nesl_utility/Simulink-PS Converter  PhysicalDomain=network_engine_domain  SubClassName=ps_input  LeftPortType=input  RightPortType=output  PseudoPeriodic=off  Frequencies=[]  NoiseDistribution=none  NoiseParameters=[]  Unit=kg/s  AffineConversion=off  FilteringAndDerivatives=provide  SimscapeFilterOrder=1  InputFilterTimeConstant=0.001  UdotUserProvided=0
  SL_PS_ProdV6 : nesl_utility/Simulink-PS Converter  PhysicalDomain=network_engine_domain  SubClassName=ps_input  LeftPortType=input  RightPortType=output  PseudoPeriodic=off  Frequencies=[]  NoiseDistribution=none  NoiseParameters=[]  Unit=kg/s  AffineConversion=off  FilteringAndDerivatives=provide  SimscapeFilterOrder=1  InputFilterTimeConstant=0.001  UdotUserProvided=0
  SL_PS_Prod_V2_ToFillingLine3V : nesl_utility/Simulink-PS Converter  PhysicalDomain=network_engine_domain  SubClassName=ps_input  LeftPortType=input  RightPortType=output  PseudoPeriodic=off  Frequencies=[]  NoiseDistribution=none  NoiseParameters=[]  Unit=1  AffineConversion=off  FilteringAndDerivatives=provide  SimscapeFilterOrder=1  InputFilterTimeConstant=0.001  UdotUserProvided=0
  SL_PS_V001 : nesl_utility/Simulink-PS Converter  PhysicalDomain=network_engine_domain  SubClassName=ps_input  LeftPortType=input  RightPortType=output  PseudoPeriodic=off  Frequencies=[]  NoiseDistribution=none  NoiseParameters=[]  Unit=1  AffineConversion=off  FilteringAndDerivatives=provide  SimscapeFilterOrder=1  InputFilterTimeConstant=0.001  UdotUserProvided=0
  SL_PS_V2 : nesl_utility/Simulink-PS Converter  PhysicalDomain=network_engine_domain  SubClassName=ps_input  LeftPortType=input  RightPortType=output  PseudoPeriodic=off  Frequencies=[]  NoiseDistribution=none  NoiseParameters=[]  Unit=1  AffineConversion=off  FilteringAndDerivatives=provide  SimscapeFilterOrder=1  InputFilterTimeConstant=0.001  UdotUserProvided=0
  Scope_M1_Angle : Scope  NumInputPorts=2
      settings: ActiveDisplayYMinimum=-20026.556036849826  ActiveDisplayYMaximum=180239.00433164847  DataLoggingVariableName=ScopeData4
  Scope_M1_RPM : Scope  NumInputPorts=2
      settings: ActiveDisplayYMinimum=-98.481117602879  ActiveDisplayYMaximum=886.33005842591126  DataLoggingVariableName=ScopeData5
  Scope_TK1_Level and Volum : Scope  NumInputPorts=3
      settings: ActiveDisplayYMinimum=-0.74999999999999978  ActiveDisplayYMaximum=6.75  DataLoggingVariableName=ScopeData7
  Scope_TK1_Temp1 : Scope  NumInputPorts=2
      settings: ActiveDisplayYMinimum=297.33962026109123  ActiveDisplayYMaximum=301.11008431684564  DataLoggingVariableName=ScopeData10
  Scope_TK1_gaugePressure : Scope  NumInputPorts=2
      settings: ActiveDisplayYMinimum=-38774.766423074929  ActiveDisplayYMaximum=-26907.823544143368  DataLoggingVariableName=ScopeData11
  Solver Configuration : nesl_utility/Solver Configuration  PhysicalDomain=network_engine_domain  SubClassName=solver  LeftPortType=input  RightPortType=generic  Tones=[]  Harmonics=[]  SimulateNoise=off  Profile=off  UseLocalSampling=off  EnableSwitchedLinearOptims=on  FrequencyDomain=off  UseCCode=off  RelTol=0.001  AbsTol=0.001  MinStep=1e-09  ToWorkspace=off  RevertToSquareIcSolve=off  NumHomotopyIterations=100  PhasorMode=off  PhasorModeNumHarmonics=1  ConsistencySolver=NEWTON_XTOL_AFTER_FTOL  IndexReductionMethod=DerivativeReplacement  DoDC=off  ResidualTolerance=1e-09  ConsistencyTolSource=GLOBAL  ConsistencyAbsTol=0.001  ConsistencyRelTol=0.001  ConsistencyTolFactor=0.1  UseLocalSolver=on  LocalSolverChoice=NE_BACKWARD_EULER_ADVANCER  ResolveIndetEquations=on  FunctionEvalNumThread=1  LocalSolverSampleTime=0.005  DoFixedCost=off  MaxNonlinIter=3  MaxModeIter=2  ComputeImpulses=off  ImpulseIterations=2  LinearAlgebra=auto  LinearAlgebraNumThread=0  EquationFormulation=NE_TIME_EF  DelaysMemoryBudget=1024  AutomaticFiltering=on  FilteringTimeConstant=0.001  PartitionStorageMethod=AS_NEEDED  PartitionMemoryBudget=1024  PartitionMethod=ROBUST  MultibodyUseLocalSolver=off  MultibodyLocalSolverChoice=ODE1  MultibodyLocalSolverSampleTime=0.001
  Sum{,1..9} (10 alike) : Sum  Inputs=|++
  TK1 : SimscapeFluids_lib/Thermal Liquid/Tanks & Accumulators/Tank (TL)  num_inlet=fluids.thermal_liquid.tanks_accumulators.enum.NumInlet.Two  pressure_spec=fluids.thermal_liquid.tanks_accumulators.enum.TankPressureSpec.Atmospheric  tank_pressure=0.101325 MPa  volume_spec=fluids.thermal_liquid.tanks_accumulators.enum.TankVolumeSpec.Constant  tank_area=1.24 m^2  level_TLU=[0, 3, 5] m  volume_TLU=[0, 4, 6] m^3  inlet_height_A=0.1 m  inlet_area_A=0.01 m^2  inlet_heights_AB=[0.02, 0.02] m  inlet_areas_AB=[0.01, 0.01] m^2  inlet_heights_ABC=[.1, .1, .1] m  inlet_areas_ABC=[.01, .01, .01] m^2  inlet_heights_ABCD=0.1 * ones(1, 4) m  inlet_areas_ABCD=0.01 * ones(1, 4) m^2  inlet_heights_ABCDE=0.1 * ones(1, 5) m  inlet_areas_ABCDE=0.01 * ones(1, 5) m^2  inlet_heights_ABCDEF=0.1 * ones(1, 6) m  inlet_areas_ABCDEF=0.01 * ones(1, 6) m^2  level_check=simscape.enum.assert.action.warn  capacity_check=simscape.enum.assert.action.none  max_capacity=10 m^3  g=9.81 m/s^2  level_specify=on  level_priority=High  level=0.2 m  level_nominal_specify=on  level_nominal_value=2  level_nominal_unit=m  volume_specify=off  volume_priority=None  volume=5 m^3  volume_nominal_specify=off  volume_nominal_value=2  volume_nominal_unit=m^3  mass_specify=off  mass_priority=None  mass=5000 kg  mass_nominal_specify=off  mass_nominal_value=1  mass_nominal_unit=kg  T_I_specify=on  T_I_priority=Low  T_I=300 K  T_I_nominal_specify=off  T_I_nominal_value=1  T_I_nominal_unit=K
      settings: InternalSimscapePortConfiguration="{\"Bottom\":[{\"id\":\"H\",\"label\":\"H\",\"type\":\"foundation.thermal.thermal\"},{\"id\":\"T_out\",\"label\":\"T\",\"type\":\"output\"}],\"Left\":[{\"id\":\"A\",\"label\":\"A\",\"type\":\"foundation.thermal_liquid.thermal_liquid\"},{\"id\":\"B\",\"label\":\"B\",\"type\":\"foundation.thermal_liquid.thermal_liquid\"}],\"Right\":[],\"Top\":[{\"id\":\"V_out\",\"label\":\"V\",\"type\":\"output\"},{\"id\":\"L_out\",\"label\":\"L\",\"type\":\"output\"}]}"
  Thermal Reference : fl_lib/Thermal/Thermal Elements/Thermal Reference
  To Workspace1 : ToWorkspace  VariableName=MassFlowRateProd  SaveFormat=Timeseries  SampleTime=-1
  To Workspace10 : ToWorkspace  VariableName=MassFlowRateCIPDischarge  SaveFormat=Timeseries  SampleTime=-1
  To Workspace11 : ToWorkspace  VariableName=MassFlowRateProdDischarge  SaveFormat=Timeseries  SampleTime=-1
  To Workspace2 : ToWorkspace  VariableName=TemperatureOut  SaveFormat=Timeseries  SampleTime=-1
  To Workspace3 : ToWorkspace  VariableName=M1_RPM  SaveFormat=Timeseries  SampleTime=-1
  To Workspace4 : ToWorkspace  VariableName=M1_Angle  SaveFormat=Timeseries  SampleTime=-1
  To Workspace5 : ToWorkspace  VariableName=TK1_pressure  SaveFormat=Timeseries  SampleTime=-1
  To Workspace6 : ToWorkspace  VariableName=TK1_Level  SaveFormat=Timeseries  SampleTime=-1
  To Workspace7 : ToWorkspace  VariableName=TK1_Volume  SaveFormat=Timeseries  SampleTime=-1
  To Workspace8 : ToWorkspace  VariableName=TK1_Temp  SaveFormat=Timeseries  SampleTime=-1
  To Workspace9 : ToWorkspace  VariableName=MassFlowRateCIP  SaveFormat=Timeseries  SampleTime=-1
  V001_InletValve : fl_lib/Thermal Liquid/Elements/Local Restriction (TL)  restriction_type=foundation.enum.restriction_type.variable  restriction_area=0.001 m^2  min_area=1e-10 m^2  max_area=0.005 m^2  area=0.01 m^2  Cd=0.64  Re_c=150  pressure_recovery=true
      settings: InternalSimscapePortConfiguration="{\"Bottom\":[],\"Left\":[{\"id\":\"A\",\"label\":\"A\",\"type\":\"foundation.thermal_liquid.thermal_liquid\"},{\"id\":\"area_in\",\"label\":\"AR\",\"type\":\"input\"}],\"Right\":[{\"id\":\"B\",\"label\":\"B\",\"type\":\"foundation.thermal_liquid.thermal_liquid\"}],\"Top\":[]}"
  VST2V4 : nesl_utility/Simulink-PS Converter  PhysicalDomain=network_engine_domain  SubClassName=ps_input  LeftPortType=input  RightPortType=output  PseudoPeriodic=off  Frequencies=[]  NoiseDistribution=none  NoiseParameters=[]  Unit=J/s  AffineConversion=off  FilteringAndDerivatives=provide  SimscapeFilterOrder=1  InputFilterTimeConstant=0.001  UdotUserProvided=0
  Volume Chamber (TL) : fl_lib/Thermal Liquid/Elements/Constant Volume Chamber (TL)  Commented=on  volume=0.01 m^3  num_ports=foundation.enum.num_ports.one  area_A=0.01 m^2  area_B=0.01 m^2  area_C=0.01 m^2  area_D=0.01 m^2  p_I_specify=off  p_I_priority=Low  p_I=0.101325 MPa  p_I_nominal_specify=off  p_I_nominal_value=1  p_I_nominal_unit=MPa  T_I_specify=off  T_I_priority=Low  T_I=300 K  T_I_nominal_specify=off  T_I_nominal_value=1  T_I_nominal_unit=K  u_I_specify=off  u_I_priority=None  u_I=83.906 kJ/kg  u_I_nominal_specify=off  u_I_nominal_value=1  u_I_nominal_unit=kJ/kg  rho_I_specify=off  rho_I_priority=None  rho_I=998.21 kg/m^3  rho_I_nominal_specify=off  rho_I_nominal_value=1  rho_I_nominal_unit=kg/m^3
      settings: InternalSimscapePortConfiguration="{\"Bottom\":[],\"Left\":[{\"id\":\"A\",\"label\":\"A\",\"type\":\"foundation.thermal_liquid.thermal_liquid\"},{\"id\":\"H\",\"label\":\"H\",\"type\":\"foundation.thermal.thermal\"}],\"Right\":[],\"Top\":[]}"
  return temp : Scope  NumInputPorts=2
      settings: ActiveDisplayYMinimum=-1  ActiveDisplayYMaximum=1  DataLoggingVariableName=ScopeData8
  Level : Outport
  Temp : Outport  Port=2
  wires:
  Random Number4/1 -> Sum4/2
  "Prod_ToFillingValve "/1 -> SL_PS_Prod_V2_ToFillingLine3V/1
  Random Number2/1 -> Sum2/2
  Sum1/1 -> To Workspace8/1, Scope_TK1_Temp1/2
  PS_SL_FIT3/1 -> Sum3/1, Log_MassFlowRateProdTrue/1
  PS-Simulink Converter2/1 -> Level/1, Sum2/1
  Random Number1/1 -> Sum1/2
  Prod_InletValve/1 -> SL_PS_V001/1
  Sum3/1 -> Prod_IN_PumpFlow/2, To Workspace1/1
  Gain/1 -> VST2V4/1
  Sum/1 -> To Workspace3/1, Scope_M1_RPM/1
  Random Number6/1 -> Sum6/2
  Random Number5/1 -> Sum5/2
  " CIP_InletValve"/1 -> SL_PS_CIPV1/1
  SteamValve/1 -> Gain/1
  PS-Simulink Converter1/1 -> Temp/1, Sum1/1
  Sum5/1 -> To Workspace4/1, Scope_M1_Angle/1
  PS-Simulink Converter/1 -> Sum6/1
  Prod_ToTankValve/1 -> SL_PS_V2/1
  Sum4/1 -> Scope_TK1_gaugePressure/2, To Workspace5/1
  PS-Simulink Converter4/1 -> Sum4/1
  Prod_FillPump_NominalFlow/1 -> SL_PS_CIPV4/1
  CIP_ReturnValve/1 -> SL_PS_CIPV3/1
  Random Number/1 -> Sum/2
  Sum6/1 -> To Workspace2/1, return temp/2
  Random Number3/1 -> Sum3/2
  K_Mix_M2/1 -> Display_MixPress_TK2/1
  Sum2/1 -> To Workspace6/1, Scope_TK1_Level and Volum/3
  CIP_SupplyPump_NominalFlow/1 -> SL_PS_CIPV5/1
  Sum7/1 -> CIP_IN_PumpFlow/2, To Workspace9/1
  CIP_SL_FIT1/1 -> Sum7/1, Log_MassFlowRateCIPTrue/1
  Random Number7/1 -> Sum7/2
  PS-Simulink Converter3/1 -> Scope_TK1_Level and Volum/2, To Workspace7/1
  Random Number8/1 -> Sum8/2
  Sum8/1 -> To Workspace10/1, CIP_Discharge_PumpFlow/2
  CIP_PS_SL_FIT1/1 -> Sum8/1, Log_MassFlowRateCIPDischargeTrue/1
  Prod_PS_SL_FIT2/1 -> Sum9/1, Log_MassFlowRateProdDischargeTrue/1
  Random Number9/1 -> Sum9/2
  Sum9/1 -> Prod_Discharge_PumpFlow/2, To Workspace11/1
  Mode/1 -> CIP_IN_PumpFlow/1, Scope_TK1_Level and Volum/1, Scope_TK1_Temp1/1, Scope_TK1_gaugePressure/1, Scope_M1_Angle/2, Scope_M1_RPM/2, Prod_IN_PumpFlow/1, CIP_Discharge_PumpFlow/1, Prod_Discharge_PumpFlow/1, return temp/1
  CIP_ReturnPump_NominalFlow/1 -> SL_PS_CIPV2/1
  Prod_DischargePump_NominalFlow/1 -> SL_PS_ProdV6/1
  " AgitatorRPM"/1 -> Agitator_RO_FirstOrder/1
  Agitator_RO_FirstOrder/1 -> Agitator_RO_Saturation/1
  Agitator_RO_Saturation/1 -> Agitator_RO_RPM_to_RadS/1, Sum/1, Log_AgitatorSpeedTrueRPM/1
  Agitator_RO_RPM_to_RadS/1 -> Agitator_RO_AngleIntegrator/1, K_Mix_M2/1
  Agitator_RO_AngleIntegrator/1 -> Sum5/1, Log_AgitatorAngleTrueRad/1
  Prod_FillFlowCmd/1 -> Prod_FillPump_CommandDynamics/1, Prod_FillPump_NominalFlow/1, Log_v46_prod_fill_cmd/1
  Prod_FillPump_CommandDynamics/1 -> Prod_FillPump_CommandDynamics_Saturation/1
  Prod_FillPump_CommandDynamics_Saturation/1 -> Log_eff_prod_fill_pump_cmd/1
  Prod_DischargeFlowCmd/1 -> Prod_DischargePump_CommandDynamics/1, Prod_DischargePump_NominalFlow/1, Log_v46_prod_discharge_cmd/1
  Prod_DischargePump_CommandDynamics/1 -> Prod_DischargePump_CommandDynamics_Saturation/1
  Prod_DischargePump_CommandDynamics_Saturation/1 -> Log_eff_prod_discharge_pump_cmd/1
  CIP_SupplyFlowCmd/1 -> CIP_SupplyPump_CommandDynamics/1, CIP_SupplyPump_NominalFlow/1, Log_v46_cip_supply_cmd/1
  CIP_SupplyPump_CommandDynamics/1 -> CIP_SupplyPump_CommandDynamics_Saturation/1
  CIP_SupplyPump_CommandDynamics_Saturation/1 -> Log_eff_cip_supply_pump_cmd/1
  CIP_ReturnFlowCmd/1 -> CIP_ReturnPump_CommandDynamics/1, CIP_ReturnPump_NominalFlow/1, Log_v46_cip_return_cmd/1
  CIP_ReturnPump_CommandDynamics/1 -> CIP_ReturnPump_CommandDynamics_Saturation/1
  CIP_ReturnPump_CommandDynamics_Saturation/1 -> Log_eff_cip_return_pump_cmd/1
  connections:
  TK1/LConn2 -- Prod_V2_ToFillingLine3/LConn1 -- CIP_V3_ReturnValve/LConn1
  CIP_Return_Drain/LConn1 -- FIT1_FlowSensor3/RConn1 -- Pressure & Temperature Sensor (TL)/LConn1
  Volume Chamber (TL)/LConn2 -- Controlled Heat Flow Rate Source/LConn1 -- TK1/RConn1
  PS_P1_FlowSource/LConn1 -- V001_InletValve/RConn1
  Solver Configuration/RConn1 -- FIT1_FlowSensor4/RConn1 -- FillingLine_Outlet/LConn1 -- Fluid_Properties_or_Settings1/RConn1
  PS_V2_ToTanksValve/RConn1 -- Pressure & Temperature Sensor (TL)1/LConn1 -- TK1/LConn1
  PSPipeFlow Resistance (TL)/RConn1 -- PS_V2_ToTanksValve/LConn1
  SL_PS_V2/RConn1 -- PS_V2_ToTanksValve/LConn2
  Controlled Heat Flow Rate Source/RConn2 -- Thermal Reference/LConn1
  SL_PS_CIPV1/RConn1 -- CIP_V1_InletValve/LConn2
  SL_PS_CIPV3/RConn1 -- CIP_V3_ReturnValve/LConn2
  SL_PS_Prod_V2_ToFillingLine3V/RConn1 -- Prod_V2_ToFillingLine3/LConn2
  AgitatorSS_M1/LConn1 -- Volume Chamber (TL)/LConn1
  PS_SL_FIT3/LConn1 -- FIT1_FlowSensor1/RConn2
  CIP_RP_FlowSource/RConn1 -- CIPPipeFlow Resistance (TL) drain/RConn1
  CIP_RP_FlowSource/LConn1 -- CIP_V3_ReturnValve/RConn1
  Pressure & Temperature Sensor (TL)/RConn1 -- PS-Simulink Converter/LConn1
  TK1/RConn2 -- PS-Simulink Converter1/LConn1
  FIT1_FlowSensor1/RConn1 -- FIT1_FlowSensor2/RConn1 -- PSPipeFlow Resistance (TL)/LConn1
  SL_PS_V001/RConn1 -- V001_InletValve/LConn2
  VST2V4/RConn1 -- Controlled Heat Flow Rate Source/RConn1
  CIP_RP_FlowSource/LConn2 -- SL_PS_CIPV2/RConn1
  PS-Simulink Converter3/LConn1 -- TK1/LConn3
  PS_P1_FlowSource/RConn1 -- FIT1_FlowSensor1/LConn1
  PS-Simulink Converter4/LConn1 -- Pressure & Temperature Sensor (TL)1/RConn1
  SL_PS_CIPV4/RConn1 -- PS_P1_FlowSource/LConn2
  PS-Simulink Converter2/LConn1 -- TK1/LConn4
  Raw_Product_Source/LConn1 -- V001_InletValve/LConn1
  CIP_Supply/LConn1 -- CIP_V1_InletValve/LConn1
  SL_PS_CIPV5/RConn1 -- CIP_P_FlowSource2/LConn2
  CIP_V1_InletValve/RConn1 -- CIP_P_FlowSource2/LConn1
  CIP_SL_FIT1/LConn1 -- FIT1_FlowSensor2/RConn2
  CIP_P_FlowSource2/RConn1 -- FIT1_FlowSensor2/LConn1
  Prod_RP_FlowSource/RConn1 -- ProdPipeFlow Resistance (TL) drain/RConn1
  Prod_RP_FlowSource/LConn2 -- SL_PS_ProdV6/RConn1
  Prod_V2_ToFillingLine3/RConn1 -- Prod_RP_FlowSource/LConn1
  CIP_PS_SL_FIT1/LConn1 -- FIT1_FlowSensor3/RConn2
  CIPPipeFlow Resistance (TL) drain/LConn1 -- FIT1_FlowSensor3/LConn1
  Prod_PS_SL_FIT2/LConn1 -- FIT1_FlowSensor4/RConn2
  ProdPipeFlow Resistance (TL) drain/LConn1 -- FIT1_FlowSensor4/LConn1
